simulink model "Model_MapPID_VDBTire"  (R2023a)
settings: Solver=VariableStepAuto  StartTime=0.0  StopTime=10  MaxStep=0.002  RelTol=1e-6
undefined symbols (not defined in the file): act_gain_mult, c, C_alpha_f, C_col, ctrl_delay, DiscIntNeverNeededParam, e_p0, F_zf, Iz, J_col, K, l_f, l_r, m, MapPID_H_den, MapPID_H_num, MapPID_Kaw, MapPID_Kd, MapPID_Ki, MapPID_Kp, MapPID_table, MapPID_Tf, MapPID_Ts_bp, MapPID_Ts_ctrl, MapPID_v_bp, motor_wm, n_st, noise_seed_a_y, noise_seed_gamma, noise_seed_T_s, noise_seed_theta1, noise_seed_theta2_dot, noise_seed_v, noise_var_a_y, noise_var_gamma, noise_var_T_s, noise_var_theta1, noise_var_theta2_dot, noise_var_v, sens_Tupd_a_y, sens_Tupd_gamma, sens_Tupd_T_s, sens_Tupd_theta1, sens_Tupd_theta2_dot, sens_Tupd_v, sensors_on, t_0, T_f, Tamax_table, Tamax_v_bp_ms, Tdref_ay_bp_ms2, Tdref_table, Tdref_v_bp_ms, vdb_v0
libraries: vehdynlibtire x2
settings Model: Creator=Tan_Tram  LastModifiedBy=Tan_Tram
settings DataIOCC: ReturnWorkspaceOutputs=off

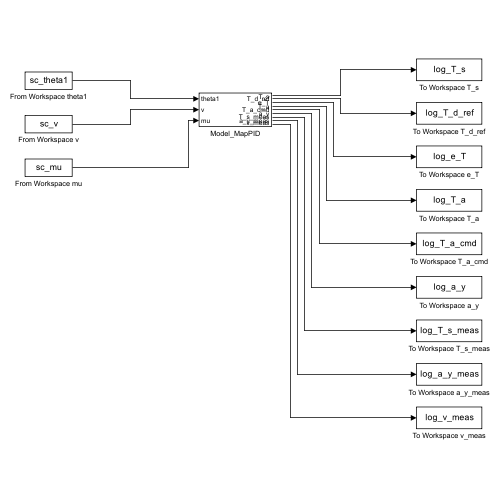
[thumbnail: Simulink's stored preview of the top-level diagram]
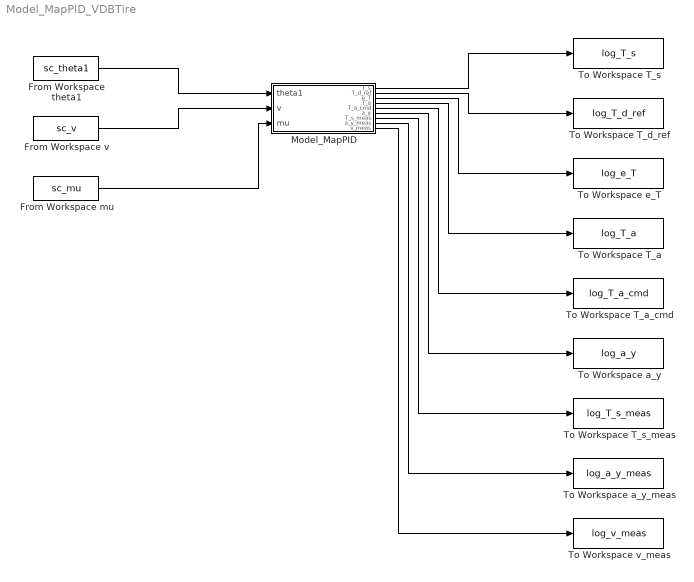
== system Model_MapPID_VDBTire ==
  From Workspace mu : FromWorkspace  VariableName=sc_mu  OutputAfterFinalValue=Holding final value
  From Workspace theta1 : FromWorkspace  VariableName=sc_theta1  OutputAfterFinalValue=Holding final value
  From Workspace v : FromWorkspace  VariableName=sc_v  OutputAfterFinalValue=Holding final value
  Model_MapPID : Subsystem
  To Workspace T_a : ToWorkspace  VariableName=log_T_a  SaveFormat=Timeseries  SampleTime=-1
  To Workspace T_a_cmd : ToWorkspace  VariableName=log_T_a_cmd  SaveFormat=Timeseries  SampleTime=-1
  To Workspace T_d_ref : ToWorkspace  VariableName=log_T_d_ref  SaveFormat=Timeseries  SampleTime=-1
  To Workspace T_s : ToWorkspace  VariableName=log_T_s  SaveFormat=Timeseries  SampleTime=-1
  To Workspace T_s_meas : ToWorkspace  VariableName=log_T_s_meas  SaveFormat=Timeseries  SampleTime=-1
  To Workspace a_y : ToWorkspace  VariableName=log_a_y  SaveFormat=Timeseries  SampleTime=-1
  To Workspace a_y_meas : ToWorkspace  VariableName=log_a_y_meas  SaveFormat=Timeseries  SampleTime=-1
  To Workspace e_T : ToWorkspace  VariableName=log_e_T  SaveFormat=Timeseries  SampleTime=-1
  To Workspace v_meas : ToWorkspace  VariableName=log_v_meas  SaveFormat=Timeseries  SampleTime=-1
  wires:
  From Workspace theta1/1 -> Model_MapPID/1(theta1)
  From Workspace v/1 -> Model_MapPID/2(v)
  From Workspace mu/1 -> Model_MapPID/3(mu)
  Model_MapPID/1(T_s) -> To Workspace T_s/1
  Model_MapPID/2(T_d_ref) -> To Workspace T_d_ref/1
  Model_MapPID/3(e_T) -> To Workspace e_T/1
  Model_MapPID/4(T_a) -> To Workspace T_a/1
  Model_MapPID/5(T_a_cmd) -> To Workspace T_a_cmd/1
  Model_MapPID/6(a_y) -> To Workspace a_y/1
  Model_MapPID/7(T_s_meas) -> To Workspace T_s_meas/1
  Model_MapPID/8(a_y_meas) -> To Workspace a_y_meas/1
  Model_MapPID/9(v_meas) -> To Workspace v_meas/1

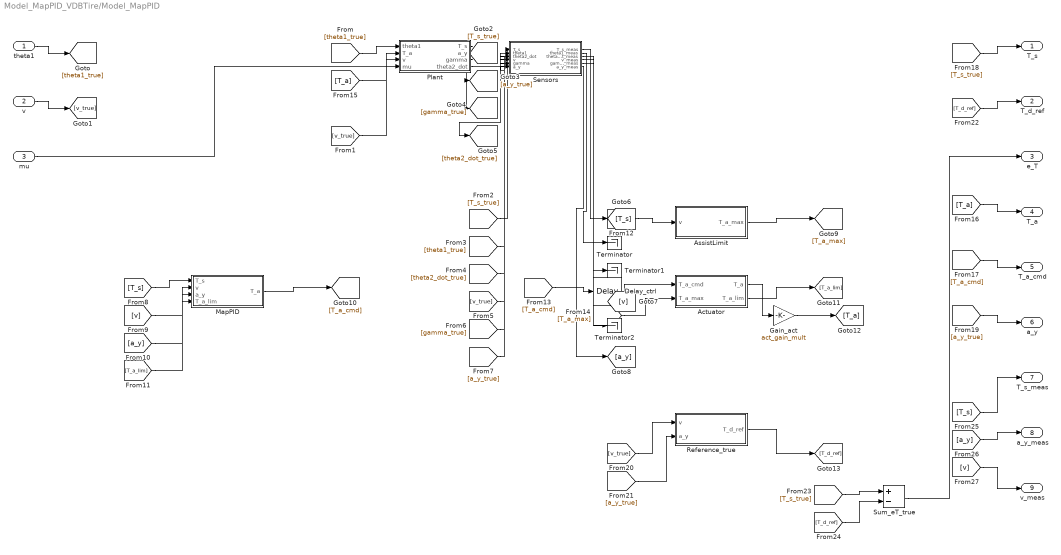
== system Model_MapPID_VDBTire/Model_MapPID ==
  theta1 : Inport
  v : Inport  Port=2
  mu : Inport  Port=3
  Actuator : Subsystem
  AssistLimit : Subsystem
  Delay_ctrl : TransportDelay  DelayTime=ctrl_delay
  Gain_act : Gain  Gain=act_gain_mult
  MapPID : Subsystem
  Plant : Subsystem
  Reference_true : Subsystem
  Sensors : Subsystem
  Sum_eT_true : Sum  Inputs=+-
  Terminator : Terminator
  Terminator1 : Terminator
  Terminator2 : Terminator
  T_s : Outport
  T_d_ref : Outport  Port=2
  e_T : Outport  Port=3
  T_a : Outport  Port=4
  T_a_cmd : Outport  Port=5
  a_y : Outport  Port=6
  T_s_meas : Outport  Port=7
  a_y_meas : Outport  Port=8
  v_meas : Outport  Port=9
  wires:
  theta1/1 -> [theta1_true]
  v/1 -> [v_true]
  mu/1 -> Plant/4(mu)
  [theta1_true] -> Plant/1(theta1)
  [v_true] -> Plant/3(v)
  Plant/1(T_s) -> [T_s_true]
  Plant/2(a_y) -> [a_y_true]
  Plant/3(gamma) -> [gamma_true]
  Plant/4(theta2_dot) -> [theta2_dot_true]
  [T_s_true] -> Sensors/1(T_s)
  [theta1_true] -> Sensors/2(theta1)
  [theta2_dot_true] -> Sensors/3(theta2_dot)
  [v_true] -> Sensors/4(v)
  [gamma_true] -> Sensors/5(gamma)
  [a_y_true] -> Sensors/6(a_y)
  Sensors/1(T_s_meas) -> [T_s]
  Sensors/2(theta1_meas) -> Terminator/1
  Sensors/3(theta2_dot_meas) -> Terminator1/1
  Sensors/4(v_meas) -> [v]
  Sensors/5(gamma_meas) -> Terminator2/1
  Sensors/6(a_y_meas) -> [a_y]
  [T_s] -> MapPID/1(T_s)
  [v] -> MapPID/2(v)
  [a_y] -> MapPID/3(a_y)
  [T_a_lim] -> MapPID/4(T_a_lim)
  [v] -> AssistLimit/1(v)
  AssistLimit/1(T_a_max) -> [T_a_max]
  MapPID/1(T_a) -> [T_a_cmd]
  [T_a_cmd] -> Delay_ctrl/1
  Delay_ctrl/1 -> Actuator/1(T_a_cmd)
  [T_a_max] -> Actuator/2(T_a_max)
  Actuator/2(T_a_lim) -> [T_a_lim]
  Actuator/1(T_a) -> Gain_act/1
  Gain_act/1 -> [T_a]
  [T_a] -> Plant/2(T_a)
  [T_a] -> T_a/1
  [T_a_cmd] -> T_a_cmd/1
  [T_s_true] -> T_s/1
  [a_y_true] -> a_y/1
  [v_true] -> Reference_true/1(v)
  [a_y_true] -> Reference_true/2(a_y)
  Reference_true/1(T_d_ref) -> [T_d_ref]
  [T_d_ref] -> T_d_ref/1
  [T_s_true] -> Sum_eT_true/1
  [T_d_ref] -> Sum_eT_true/2
  Sum_eT_true/1 -> e_T/1
  [T_s] -> T_s_meas/1
  [a_y] -> a_y_meas/1
  [v] -> v_meas/1

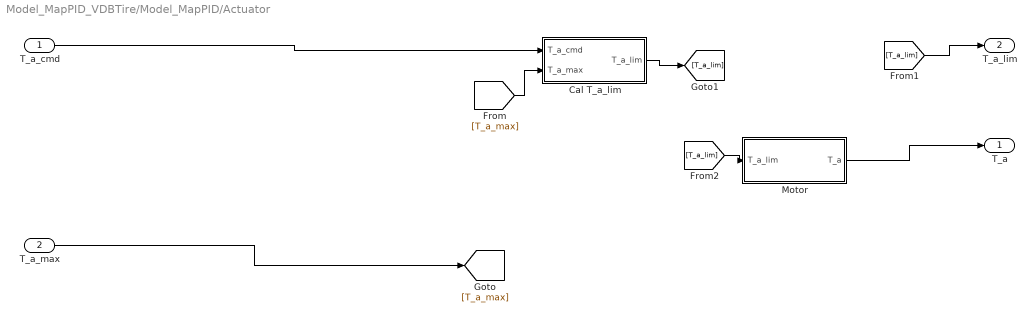
== system Model_MapPID_VDBTire/Model_MapPID/Actuator ==
  T_a_cmd : Inport
  T_a_max : Inport  Port=2
  Cal T_a_lim : Subsystem
  Motor : Subsystem
  T_a : Outport
  T_a_lim : Outport  Port=2
  wires:
  Motor/1(T_a) -> T_a/1
  [T_a_lim] -> Motor/1(T_a_lim)
  [T_a_lim] -> T_a_lim/1
  Cal T_a_lim/1(T_a_lim) -> [T_a_lim]
  [T_a_max] -> Cal T_a_lim/2(T_a_max)
  T_a_cmd/1 -> Cal T_a_lim/1(T_a_cmd)
  T_a_max/1 -> [T_a_max]

== system Model_MapPID_VDBTire/Model_MapPID/AssistLimit ==
  v : Inport
  Lookup_Tamax : Lookup_n-D  NumberOfTableDimensions=1  BreakpointsForDimension1=Tamax_v_bp_ms  Table=Tamax_table  ExtrapMethod=Clip  InternalRulePriority=Speed  RndMeth=Simplest
  T_a_max : Outport
  wires:
  Lookup_Tamax/1 -> T_a_max/1
  v/1 -> Lookup_Tamax/1

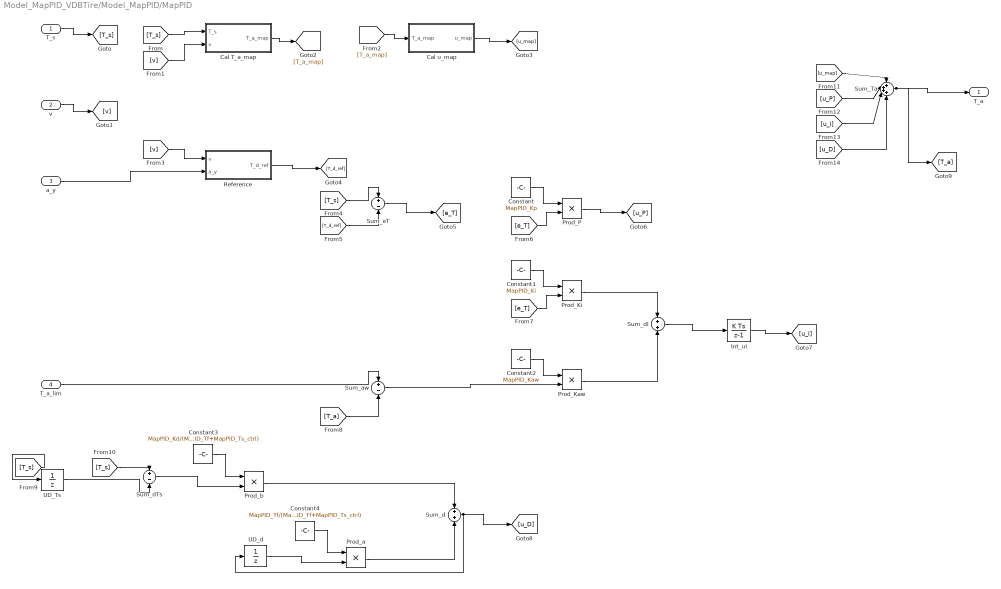
== system Model_MapPID_VDBTire/Model_MapPID/MapPID ==
  T_s : Inport
  v : Inport  Port=2
  a_y : Inport  Port=3
  T_a_lim : Inport  Port=4
  Cal T_a_map : Subsystem
  Cal u_map : Subsystem
  Constant : Constant  Value=MapPID_Kp
  Constant1 : Constant  Value=MapPID_Ki
  Constant2 : Constant  Value=MapPID_Kaw
  Constant3 : Constant  Value=MapPID_Kd/(MapPID_Tf+MapPID_Ts_ctrl)
  Constant4 : Constant  Value=MapPID_Tf/(MapPID_Tf+MapPID_Ts_ctrl)
  Int_uI : DiscreteIntegrator  gainval=1  SampleTime=MapPID_Ts_ctrl  ICPrevOutput=DiscIntNeverNeededParam  ICPrevScaledInput=DiscIntNeverNeededParam
  Prod_Kaw : Product  Inputs=**
  Prod_Ki : Product  Inputs=**
  Prod_P : Product  Inputs=**
  Prod_a : Product  Inputs=**
  Prod_b : Product  Inputs=**
  Reference : Subsystem
  Sum_Ta : Sum  Inputs=++++
  Sum_aw : Sum  Inputs=+-
  Sum_d : Sum
  Sum_dI : Sum
  Sum_dTs : Sum  Inputs=+-
  Sum_eT : Sum  Inputs=+-
  UD_Ts : UnitDelay  SampleTime=MapPID_Ts_ctrl  HasFrameUpgradeWarning=on
  UD_d : UnitDelay  SampleTime=MapPID_Ts_ctrl  HasFrameUpgradeWarning=on
  T_a : Outport
  wires:
  Sum_Ta/1 -> [T_a], T_a/1
  [u_D] -> Sum_Ta/4
  [u_I] -> Sum_Ta/3
  [u_P] -> Sum_Ta/2
  [u_map] -> Sum_Ta/1
  Sum_d/1 -> [u_D], UD_d/1
  Prod_a/1 -> Sum_d/2
  Prod_b/1 -> Sum_d/1
  UD_d/1 -> Prod_a/2
  Constant4/1 -> Prod_a/1
  Sum_dTs/1 -> Prod_b/2
  Constant3/1 -> Prod_b/1
  UD_Ts/1 -> Sum_dTs/2
  [T_s] -> Sum_dTs/1
  [T_s] -> UD_Ts/1
  Int_uI/1 -> [u_I]
  Sum_dI/1 -> Int_uI/1
  Prod_Kaw/1 -> Sum_dI/2
  Prod_Ki/1 -> Sum_dI/1
  Sum_aw/1 -> Prod_Kaw/2
  Constant2/1 -> Prod_Kaw/1
  [T_a] -> Sum_aw/2
  T_a_lim/1 -> Sum_aw/1
  [e_T] -> Prod_Ki/2
  Constant1/1 -> Prod_Ki/1
  Prod_P/1 -> [u_P]
  [e_T] -> Prod_P/2
  Constant/1 -> Prod_P/1
  Sum_eT/1 -> [e_T]
  [T_d_ref] -> Sum_eT/2
  [T_s] -> Sum_eT/1
  Reference/1(T_d_ref) -> [T_d_ref]
  a_y/1 -> Reference/2(a_y)
  [v] -> Reference/1(v)
  Cal u_map/1(u_map) -> [u_map]
  [T_a_map] -> Cal u_map/1(T_a_map)
  Cal T_a_map/1(T_a_map) -> [T_a_map]
  [v] -> Cal T_a_map/2(v)
  [T_s] -> Cal T_a_map/1(T_s)
  v/1 -> [v]
  T_s/1 -> [T_s]

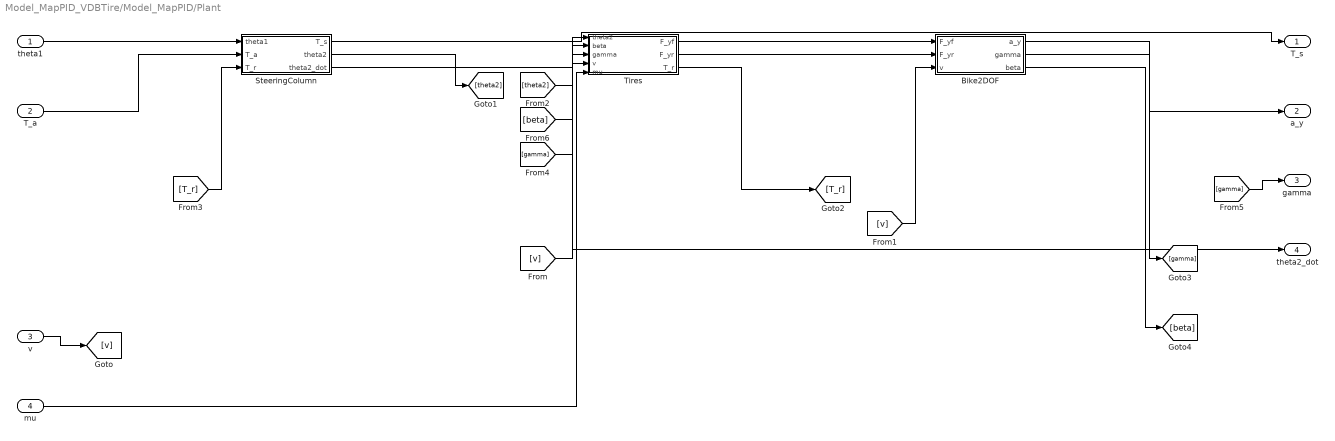
== system Model_MapPID_VDBTire/Model_MapPID/Plant ==
  theta1 : Inport
  T_a : Inport  Port=2
  v : Inport  Port=3
  mu : Inport  Port=4
  Bike2DOF : Subsystem
  SteeringColumn : Subsystem
  Tires : Subsystem
  T_s : Outport
  a_y : Outport  Port=2
  gamma : Outport  Port=3
  theta2_dot : Outport  Port=4
  wires:
  theta1/1 -> SteeringColumn/1(theta1)
  T_a/1 -> SteeringColumn/2(T_a)
  mu/1 -> Tires/5(mu)
  Tires/1(F_yf) -> Bike2DOF/1(F_yf)
  Tires/2(F_yr) -> Bike2DOF/2(F_yr)
  SteeringColumn/1(T_s) -> T_s/1
  Bike2DOF/1(a_y) -> a_y/1
  SteeringColumn/3(theta2_dot) -> theta2_dot/1
  v/1 -> [v]
  [v] -> Tires/4(v)
  [v] -> Bike2DOF/3(v)
  SteeringColumn/2(theta2) -> [theta2]
  [theta2] -> Tires/1(theta2)
  Tires/3(T_r) -> [T_r]
  [T_r] -> SteeringColumn/3(T_r)
  Bike2DOF/2(gamma) -> [gamma]
  [gamma] -> Tires/3(gamma)
  [gamma] -> gamma/1
  Bike2DOF/3(beta) -> [beta]
  [beta] -> Tires/2(beta)

== system Model_MapPID_VDBTire/Model_MapPID/Reference_true ==
  v : Inport
  a_y : Inport  Port=2
  Cal T_d_ref : Subsystem
  T_d_ref : Outport
  wires:
  Cal T_d_ref/1(T_d_ref) -> T_d_ref/1
  a_y/1 -> Cal T_d_ref/2(a_y)
  v/1 -> Cal T_d_ref/1(v)

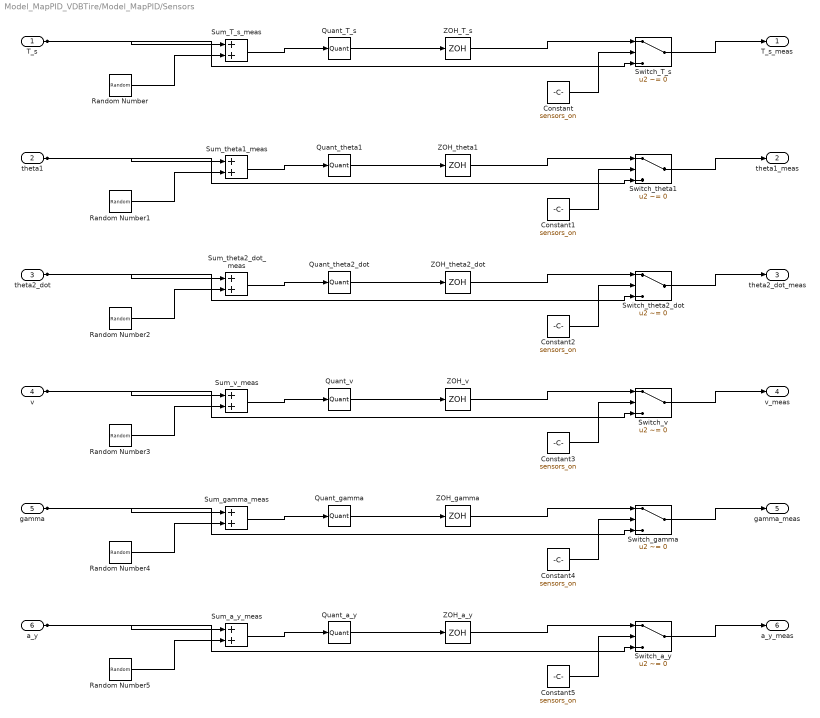
== system Model_MapPID_VDBTire/Model_MapPID/Sensors ==
  T_s : Inport
  theta1 : Inport  Port=2
  theta2_dot : Inport  Port=3
  v : Inport  Port=4
  gamma : Inport  Port=5
  a_y : Inport  Port=6
  Constant{,1..5} (6 alike) : Constant  Value=sensors_on
  Quant_T_s : Quantizer  QuantizationInterval=sens_delta_T_s
  Quant_a_y : Quantizer  QuantizationInterval=sens_delta_a_y
  Quant_gamma : Quantizer  QuantizationInterval=sens_delta_gamma
  Quant_theta1 : Quantizer  QuantizationInterval=sens_delta_theta1
  Quant_theta2_dot : Quantizer  QuantizationInterval=sens_delta_theta2_dot
  Quant_v : Quantizer  QuantizationInterval=sens_delta_v
  Random Number : RandomNumber  Variance=noise_var_T_s  Seed=noise_seed_T_s  SampleTime=sens_Tupd_T_s
  Random Number1 : RandomNumber  Variance=noise_var_theta1  Seed=noise_seed_theta1  SampleTime=sens_Tupd_theta1
  Random Number2 : RandomNumber  Variance=noise_var_theta2_dot  Seed=noise_seed_theta2_dot  SampleTime=sens_Tupd_theta2_dot
  Random Number3 : RandomNumber  Variance=noise_var_v  Seed=noise_seed_v  SampleTime=sens_Tupd_v
  Random Number4 : RandomNumber  Variance=noise_var_gamma  Seed=noise_seed_gamma  SampleTime=sens_Tupd_gamma
  Random Number5 : RandomNumber  Variance=noise_var_a_y  Seed=noise_seed_a_y  SampleTime=sens_Tupd_a_y
  Sum_T_s_meas : Sum
  Sum_a_y_meas : Sum
  Sum_gamma_meas : Sum
  Sum_theta1_meas : Sum
  Sum_theta2_dot_meas : Sum
  Sum_v_meas : Sum
  Switch_T_s : Switch  Criteria=u2 ~= 0  SaturateOnIntegerOverflow=off  InputSameDT=off
  Switch_a_y : Switch  Criteria=u2 ~= 0  SaturateOnIntegerOverflow=off  InputSameDT=off
  Switch_gamma : Switch  Criteria=u2 ~= 0  SaturateOnIntegerOverflow=off  InputSameDT=off
  Switch_theta1 : Switch  Criteria=u2 ~= 0  SaturateOnIntegerOverflow=off  InputSameDT=off
  Switch_theta2_dot : Switch  Criteria=u2 ~= 0  SaturateOnIntegerOverflow=off  InputSameDT=off
  Switch_v : Switch  Criteria=u2 ~= 0  SaturateOnIntegerOverflow=off  InputSameDT=off
  ZOH_T_s : ZeroOrderHold  SampleTime=sens_Tupd_T_s
  ZOH_a_y : ZeroOrderHold  SampleTime=sens_Tupd_a_y
  ZOH_gamma : ZeroOrderHold  SampleTime=sens_Tupd_gamma
  ZOH_theta1 : ZeroOrderHold  SampleTime=sens_Tupd_theta1
  ZOH_theta2_dot : ZeroOrderHold  SampleTime=sens_Tupd_theta2_dot
  ZOH_v : ZeroOrderHold  SampleTime=sens_Tupd_v
  T_s_meas : Outport
  theta1_meas : Outport  Port=2
  theta2_dot_meas : Outport  Port=3
  v_meas : Outport  Port=4
  gamma_meas : Outport  Port=5
  a_y_meas : Outport  Port=6
  wires:
  Switch_a_y/1 -> a_y_meas/1
  Constant5/1 -> Switch_a_y/2
  ZOH_a_y/1 -> Switch_a_y/1
  Quant_a_y/1 -> ZOH_a_y/1
  Sum_a_y_meas/1 -> Quant_a_y/1
  Random Number5/1 -> Sum_a_y_meas/2
  a_y/1 -> Switch_a_y/3, Sum_a_y_meas/1
  Switch_gamma/1 -> gamma_meas/1
  Constant4/1 -> Switch_gamma/2
  ZOH_gamma/1 -> Switch_gamma/1
  Quant_gamma/1 -> ZOH_gamma/1
  Sum_gamma_meas/1 -> Quant_gamma/1
  Random Number4/1 -> Sum_gamma_meas/2
  gamma/1 -> Switch_gamma/3, Sum_gamma_meas/1
  Switch_v/1 -> v_meas/1
  Constant3/1 -> Switch_v/2
  ZOH_v/1 -> Switch_v/1
  Quant_v/1 -> ZOH_v/1
  Sum_v_meas/1 -> Quant_v/1
  Random Number3/1 -> Sum_v_meas/2
  v/1 -> Switch_v/3, Sum_v_meas/1
  Switch_theta2_dot/1 -> theta2_dot_meas/1
  Constant2/1 -> Switch_theta2_dot/2
  ZOH_theta2_dot/1 -> Switch_theta2_dot/1
  Quant_theta2_dot/1 -> ZOH_theta2_dot/1
  Sum_theta2_dot_meas/1 -> Quant_theta2_dot/1
  Random Number2/1 -> Sum_theta2_dot_meas/2
  theta2_dot/1 -> Switch_theta2_dot/3, Sum_theta2_dot_meas/1
  Switch_theta1/1 -> theta1_meas/1
  Constant1/1 -> Switch_theta1/2
  ZOH_theta1/1 -> Switch_theta1/1
  Quant_theta1/1 -> ZOH_theta1/1
  Sum_theta1_meas/1 -> Quant_theta1/1
  Random Number1/1 -> Sum_theta1_meas/2
  theta1/1 -> Switch_theta1/3, Sum_theta1_meas/1
  Switch_T_s/1 -> T_s_meas/1
  Constant/1 -> Switch_T_s/2
  ZOH_T_s/1 -> Switch_T_s/1
  Quant_T_s/1 -> ZOH_T_s/1
  Sum_T_s_meas/1 -> Quant_T_s/1
  Random Number/1 -> Sum_T_s_meas/2
  T_s/1 -> Switch_T_s/3, Sum_T_s_meas/1

== system Model_MapPID_VDBTire/Model_MapPID/Actuator/Cal T_a_lim ==
  T_a_cmd : Inport
  T_a_max : Inport  Port=2
  Max_Ta : MinMax  Function=max  Inputs=2
  Min_Ta : MinMax  Inputs=2
  Neg_Tamax : UnaryMinus
  T_a_lim : Outport
  wires:
  Max_Ta/1 -> T_a_lim/1
  Neg_Tamax/1 -> Max_Ta/2
  Min_Ta/1 -> Max_Ta/1
  [T_a_max] -> Neg_Tamax/1
  [T_a_max] -> Min_Ta/2
  T_a_cmd/1 -> Min_Ta/1
  T_a_max/1 -> [T_a_max]

== system Model_MapPID_VDBTire/Model_MapPID/Actuator/Motor ==
  T_a_lim : Inport
  Motor_lag : TransferFcn  Numerator=[motor_wm]  Denominator=[1 motor_wm]
  T_a : Outport
  wires:
  Motor_lag/1 -> T_a/1
  T_a_lim/1 -> Motor_lag/1

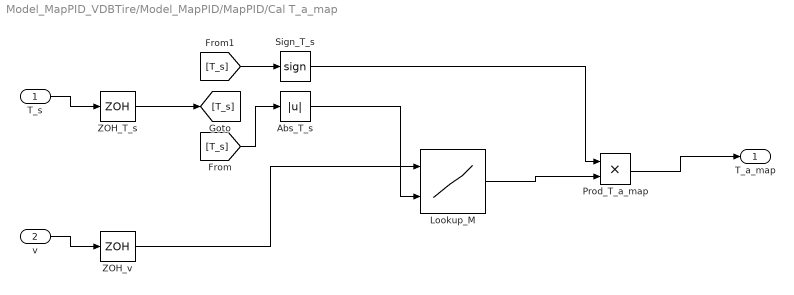
== system Model_MapPID_VDBTire/Model_MapPID/MapPID/Cal T_a_map ==
  T_s : Inport
  v : Inport  Port=2
  Abs_T_s : Abs  SaturateOnIntegerOverflow=off
  Lookup_M : Lookup_n-D  BreakpointsForDimension1=MapPID_v_bp  BreakpointsForDimension2=MapPID_Ts_bp  BreakpointsForDimension3=[5, 7]  Table=MapPID_table  ExtrapMethod=Clip  InternalRulePriority=Speed  RndMeth=Simplest
      settings: InputPortMap=u0,u1
  Prod_T_a_map : Product  Inputs=**
  Sign_T_s : Signum
  ZOH_T_s : ZeroOrderHold  SampleTime=MapPID_Ts_ctrl
  ZOH_v : ZeroOrderHold  SampleTime=MapPID_Ts_ctrl
  T_a_map : Outport
  wires:
  Prod_T_a_map/1 -> T_a_map/1
  Lookup_M/1 -> Prod_T_a_map/2
  Sign_T_s/1 -> Prod_T_a_map/1
  Abs_T_s/1 -> Lookup_M/2
  ZOH_v/1 -> Lookup_M/1
  [T_s] -> Sign_T_s/1
  [T_s] -> Abs_T_s/1
  ZOH_T_s/1 -> [T_s]
  v/1 -> ZOH_v/1
  T_s/1 -> ZOH_T_s/1

== system Model_MapPID_VDBTire/Model_MapPID/MapPID/Cal u_map ==
  T_a_map : Inport
  Disc_H : DiscreteTransferFcn  Numerator=MapPID_H_num  Denominator=MapPID_H_den  SampleTime=MapPID_Ts_ctrl
  u_map : Outport
  wires:
  Disc_H/1 -> u_map/1
  [T_a_map] -> Disc_H/1
  T_a_map/1 -> [T_a_map]

== system Model_MapPID_VDBTire/Model_MapPID/MapPID/Reference ==
  v : Inport
  a_y : Inport  Port=2
  Cal T_d_ref : Subsystem
  T_d_ref : Outport
  wires:
  v/1 -> Cal T_d_ref/1(v)
  a_y/1 -> Cal T_d_ref/2(a_y)
  Cal T_d_ref/1(T_d_ref) -> T_d_ref/1

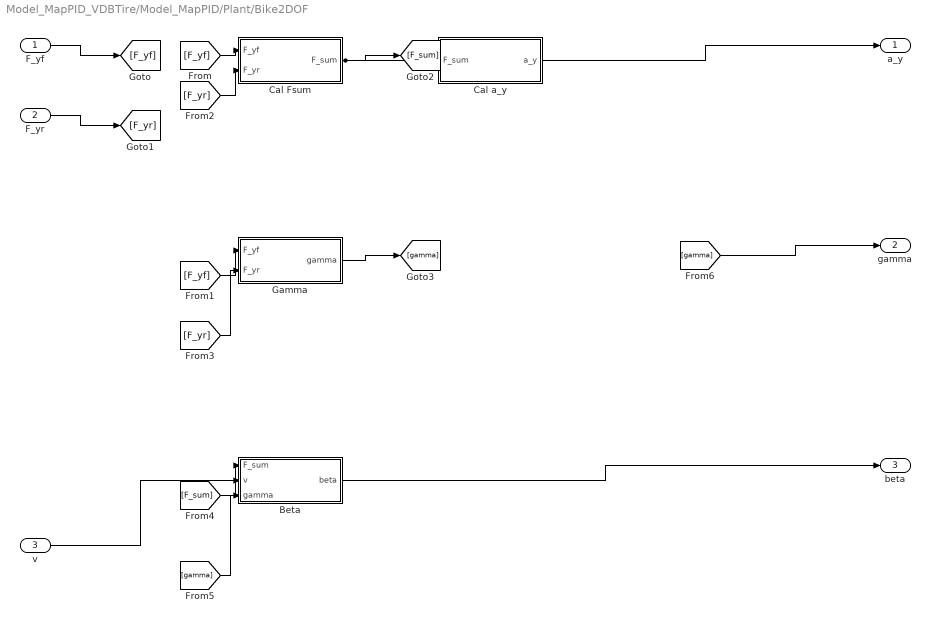
== system Model_MapPID_VDBTire/Model_MapPID/Plant/Bike2DOF ==
  F_yf : Inport
  F_yr : Inport  Port=2
  v : Inport  Port=3
  Beta : Subsystem
  Cal Fsum : Subsystem
  Cal a_y : Subsystem
  Gamma : Subsystem
  a_y : Outport
  gamma : Outport  Port=2
  beta : Outport  Port=3
  wires:
  Beta/1(beta) -> beta/1
  v/1 -> Beta/2(v)
  [gamma] -> gamma/1
  [gamma] -> Beta/3(gamma)
  Gamma/1(gamma) -> [gamma]
  Cal a_y/1(a_y) -> a_y/1
  [F_sum] -> Beta/1(F_sum)
  Cal Fsum/1(F_sum) -> [F_sum], Cal a_y/1(F_sum)
  [F_yr] -> Gamma/2(F_yr)
  [F_yr] -> Cal Fsum/2(F_yr)
  F_yr/1 -> [F_yr]
  [F_yf] -> Gamma/1(F_yf)
  [F_yf] -> Cal Fsum/1(F_yf)
  F_yf/1 -> [F_yf]

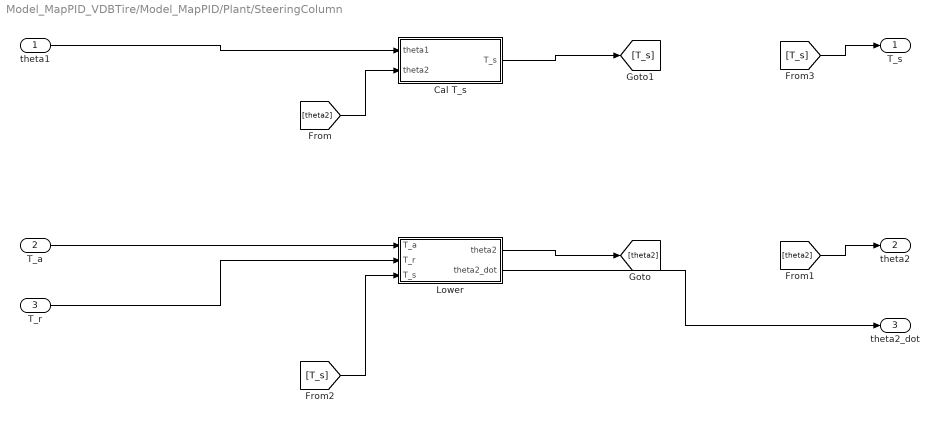
== system Model_MapPID_VDBTire/Model_MapPID/Plant/SteeringColumn ==
  theta1 : Inport
  T_a : Inport  Port=2
  T_r : Inport  Port=3
  Cal T_s : Subsystem
  Lower : Subsystem
  T_s : Outport
  theta2 : Outport  Port=2
  theta2_dot : Outport  Port=3
  wires:
  [T_s] -> T_s/1
  [T_s] -> Lower/3(T_s)
  Cal T_s/1(T_s) -> [T_s]
  [theta2] -> theta2/1
  [theta2] -> Cal T_s/2(theta2)
  Lower/1(theta2) -> [theta2]
  Lower/2(theta2_dot) -> theta2_dot/1
  T_r/1 -> Lower/2(T_r)
  T_a/1 -> Lower/1(T_a)
  theta1/1 -> Cal T_s/1(theta1)

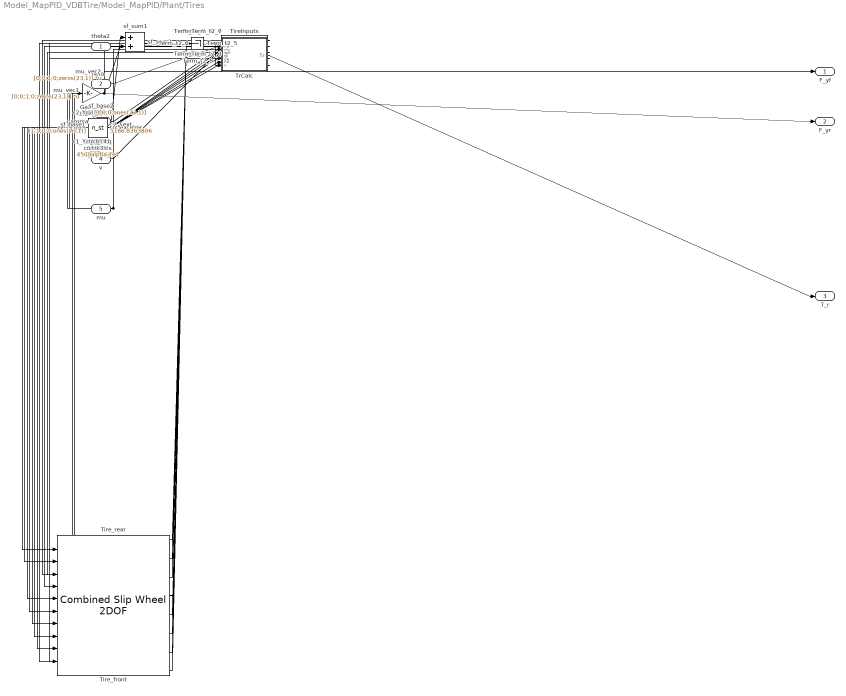
== system Model_MapPID_VDBTire/Model_MapPID/Plant/Tires ==
  theta2 : Inport
  beta : Inport  Port=2
  gamma : Inport  Port=3
  v : Inport  Port=4
  mu : Inport  Port=5
  Gain_F1 : Gain  Gain=2
  Gain_F2 : Gain  Gain=2
  Term_t1_{1..3,5..8} (7 alike) : Terminator
  Term_t2_{1..3,5..8} (7 alike) : Terminator
  TireInputs : MATLAB Function  TreatAsAtomicUnit=on
  Tire_front : vehdynlibtire/Combined Slip Wheel 2DOF  tireType=External file  BrakeType=Disc  vertType=None  plySteer=off  turnslip=off  mu_static=.3  mu_kinetic=.2  disk_abore=.05  Rm=.177  num_pads=2  drum_abore=0.0508  drum_a=0.123  drum_c=0.212  drum_r=0.15  drum_theta1=0  drum_theta2=126  brake_p_bpt=[1 11.4736842105263 21.9473684210526 32.4210526315789 42.8947368421053 53.3684210526316 63.8421052631579 74.3157894736842 84.7894736842105 95.2631578947368 105.736842105263 116.210526315789 126.684210526316 137.157894736842 147.631578947368 158.105263157895 168.578947368421 179.052631578947 189.526315789474 200]  brake_n_bpt=[0 52.6315789473684 105.263157894737 157.894736842105 210.526315789474 263.157894736842 315.789473684211 368.421052631579 421.052631578947 473.684210526316 526.315789473684 578.947368421053 631.578947368421 684.210526315789 736.842105263158 789.473684210526 842.105263157895 894.736842105263 947.368421052632 1000]  f_brake_t=[43.4900602404453 42.5056030554862 41.5350898940194 40.5780454442085 39.6340111501808 38.7025443887544 37.7832176914519 36.8756180088306 35.9793460143796 35.0940154454303 34.2192524787115 33.3546951383474 32.4999927342521 31.6548053290159 30.8188032315107 29.991666515561 29.1730845621415 28.362755623661 27.5603864089927 26.765691687993;498.991217495636 487.695866636631 476.560505099801 465.579679307235 454.748127933653 444.060772460445 433.51270824929 423.099196101319 412.81565427025 402.657650900201 392.620896861006 382.701238955775 372.894653477208 363.197240090814 353.605216024701 344.114910546964 334.722759712992 325.425301366216 316.219170376863 307.10109410434;954.492374750826 932.886130217776 911.585920305583 890.581313170261 869.862244717126 849.419000532136 829.242198807128 809.322774193808 789.651962526121 770.221286354971 751.0225412433 732.047782773203 713.289314220164 694.739674852612 676.391628817892 658.238154578366 640.272434863842 622.48784710877 604.877954344734 587.436496520688;1409.99353200602 1378.07639379892 1346.61133551136 1315.58294703329 1284.9763615006 1254.77722860383 1224.97168936497 1195.5463522863 1166.48827078199 1137.78492180974 1109.42418562559 1081.39432659063 1053.68397496312 1026.28210961441 999.178041611083 972.361398609768 945.822110014692 919.550392851325 893.536738312604 867.771898937035;1865.49468926121 1823.26665738007 1781.63675071715 1740.58458089631 1700.09047828407 1660.13545667552 1620.7011799228 1581.76993037878 1543.32457903786 1505.34855726451 1467.82583000789 1430.74087040806 1394.07863570608 1357.82454437621 1321.96445440427 1286.48464264117 1251.37178516554 1216.61293859388 1182.19552228048 1148.10730135338;2320.9958465164 2268.45692096121 2216.66216592293 2165.58621475934 2115.20459506754 2065.49368474721 2016.43067048064 1967.99350847127 1920.16088729373 1872.91219271928 1826.22747439018 1780.08741422549 1734.47329644903 1689.36697913801 1644.75086719747 1600.60788667257 1556.92146031639 1513.67548433643 1470.85430624835 1428.44270376973;2776.49700377159 2713.64718454235 2651.68758112871 2590.58784862237 2530.31871185102 2470.8519128189 2412.16016103848 2354.21708656376 2296.9971955496 2240.47582817405 2184.62911877248 2129.43395804292 2074.86795719199 2020.9094138998 1967.53727999066 1914.73113070398 1862.47113546724 1810.73803007899 1759.51309021622 1708.77810618608;3231.99816102678 3158.8374481235 3086.71299633449 3015.58948248539 2945.43282863449 2876.21014089059 2807.88965159632 2740.44066465625 2673.83350380547 2608.03946362882 2543.03076315477 2478.78050186034 2415.26261793494 2352.4518486616 2290.32369278385 2228.85437473538 2168.02081061809 2107.80057582154 2048.17187418409 1989.11350860242;3687.49931828197 3604.02771170464 3521.73841154027 3440.59111634842 3360.54694541796 3281.56836896228 3203.61914215416 3126.66424274874 3050.66981206134 2975.60309908359 2901.43240753707 2828.12704567777 2755.6572786779 2683.9942834234 2613.11010557704 2542.97761876678 2473.57048576894 2404.8631215641 2336.83065815196 2269.44891101877;4143.00047553716 4049.21797528579 3956.76382674606 3865.59275021144 3775.66106220143 3686.92659703397 3599.34863271199 3512.88782084123 3427.50612031721 3343.16673453836 3259.83405191936 3177.4735894952 3096.05193942085 3015.5367181852 2935.89651837023 2857.10086279818 2779.12016091979 2701.92566730665 2625.48944211983 2549.78431343512;4598.50163279235 4494.40823886693 4391.78924195184 4290.59438407447 4190.77517898491 4092.28482510566 3995.07812326983 3899.11139893372 3804.34242857308 3710.73036999313 3618.23569630166 3526.82013331263 3436.44660016381 3347.079152947 3258.68293116342 3171.22410682959 3084.66983607064 2998.98821304921 2914.1482260877 2830.11971585147;5054.00279004754 4939.59850244808 4826.81465715762 4715.59601793749 4605.88929576838 4497.64305317735 4390.80761382767 4285.3349770262 4181.17873682896 4078.2940054479 3976.63734068395 3876.16667713006 3776.84126090677 3678.62158770879 3581.46934395661 3485.34735086099 ...(+2764 chars)]  tireParamSet=vdynPassCar.mat  PRESMAX=1000000  PRESMIN=10000  FZMAX=28000  FZMIN=100  VXLOW=1  KPUMAX=1.5  KPUMIN=-1.5  ALPMAX=1.5  ALPMIN=-1.5  CAMMAX=0.17453  CAMMIN=-0.17453  LONGVL=16.7  FxRelFreqLwrLim=200*pi  FyRelFreqLwrLim=200*pi  MyRelFreqLwrLim=100*pi  omegao=vdb_v0/(0.97*0.5132)  br=1e-3  UNLOADED_RADIUS=0.5132  NOMPRES=793000  FNOMIN=4548.7286194  WIDTH=0.295  RIM_RADIUS=0.28575  MASS=54.96  IYY=10.664  GRAVITY=-9.81  zo=0  zdoto=0  BREFF=8.25094594147963  DREFF=0.260468730454265  FREFF=0.0735298544471851  Q_RE0=1.00866439868088  Q_V1=0.000760413786224011  Q_V2=0.0463384792019201  Q_FZ1=0  Q_FZ2=15.6870832810226  Q_FZ3=0  Q_FCX=0.138643970247602  Q_FCY=0.10843499565426  Q_FCY2=-0.465763352339538  PFZ1=0.69958166705601  VERTICAL_STIFFNESS=207885.061134007  VERTICAL_DAMPING=500  BOTTOM_OFFST=.01  BOTTOM_STIFF=2e6  LONGITUDINAL_STIFFNESS=388714.175879854  LATERAL_STIFFNESS=157087.404633332  PCFX1=0.18539229191199  PCFX2=0  PCFX3=0  PCFY1=0.163183345037677  PCFY2=0  PCFY3=0.249094918231954  Q_RA1=0.675942571700787  Q_RA2=0.73800463546164  Q_RB1=1.04487486456705  Q_RB2=-1.191763806629  PCX1=1.58523057950359  PDX1=1.0239116238178  PDX2=-0.0842405110022724  PDX3=0  PEX1=0.110312777158455  PEX2=0.313468516038146  PEX3=0  PEX4=0.0016060905760045  PKX1=21.3872544684023  PKX2=14.0006541873175  PKX3=-0.405326109653452  PHX1=0.000212599305364818  PHX2=0.00115950515263055  PVX1=1.59236164471432e-05  PVX2=0.000104321112127671  PPX1=-0.349461321276586  PPX2=0.387840040616429  PPX3=-0.0969947336569324  PPX4=0.0632271859795801  RBX1=12.7633329850276  RBX2=9.5787123658471  RBX3=0  RCX1=1.02796280922059  REX1=-0.45202516851367  REX2=-0.47304886171176  RHX1=0.000233272373115809  QSX1=-0.00788307788961443  QSX2=0.954629515459396  QSX3=0.0155855777667025  QSX4=0.125904607142414  QSX5=1.01110069703963  QSX6=20.1938577118433  QSX7=0.310818120717083  QSX8=-0.0430823751139655  QSX9=0.636494404888216  QSX10=0.142438060591663  QSX11=0.346766530036373  QSX12=0  QSX13=0  QSX14=0  PPMX1=0  PCY1=1.3  PDY1=1  PDY2=0  PDY3=0  PEY1=-1  PEY2=0  PEY3=0  PEY4=0  PEY5=0  PKY1=-17.5873319104  PKY2=1  PKY3=0  PKY4=2  PKY5=0  PKY6=0  PKY7=0  PHY1=0  PHY2=0  PVY1=0  PVY2=0  PVY3=0  PVY4=0  PPY1=0  PPY2=0  PPY3=0  PPY4=0  PPY5=0  RBY1=0  RBY2=0  RBY3=0  RBY4=0  RCY1=1  REY1=0  REY2=0  RHY1=0  RHY2=0  RVY1=0  RVY2=0  RVY3=0  RVY4=0  RVY5=0  RVY6=0  QSY1=0  QSY2=0  QSY3=0  QSY4=0  QSY5=0  QSY6=0  QSY7=0  QSY8=0  QBZ1=11.666656027484  QBZ2=-1.30355438574485  QBZ3=0  QBZ4=0.177918305399071  QBZ5=-0.162481135068033  QBZ6=0  QBZ9=30.1445534682089  QBZ10=0  QCZ1=1.29026978207574  QDZ1=0.0886972644991399  QDZ2=-0.0058634820161856  QDZ3=0.3805597481383  QDZ4=0  QDZ6=0.00160914918118959  QDZ7=-0.00211036330862154  QDZ8=-0.13921904912557  QDZ9=0.00816585550028243  QDZ10=0  QDZ11=0  QEZ1=-2.19802254534746  QEZ2=1.01850535789165  QEZ3=0  QEZ4=0.278379679112054  QEZ5=-0.548414722765386  QHZ1=0.00148361198869669  QHZ2=0.00202017567585904  QHZ3=0.240316641332066  QHZ4=-0.210114035738085  PPZ1=-0.443927982388615  PPZ2=0  SSZ1=0.00914999585397887  SSZ2=0.0389830656052735  SSZ3=0  SSZ4=0  PDXP1=0.396718274678791  PDXP2=0  PDXP3=0  PKYP1=1.00587060633573  PDYP1=0.40483048923438  PDYP2=0  PDYP3=0  PDYP4=0  PHYP1=0.992731942067188  PHYP2=0.150352945499914  PHYP3=0  PHYP4=-3.98988682633674  PECP1=0.502379254513503  PECP2=0  QDTP1=10.0178654287947  QCRP1=0.200627747200702  QCRP2=0.0995735881599772  QBRP1=0.0997107127960717  QDRP1=1.01432910167423  QDRP2=0  aMode=2
  Tire_rear : vehdynlibtire/Combined Slip Wheel 2DOF  tireType=External file  BrakeType=Disc  vertType=None  plySteer=off  turnslip=off  mu_static=.3  mu_kinetic=.2  disk_abore=.05  Rm=.177  num_pads=2  drum_abore=0.0508  drum_a=0.123  drum_c=0.212  drum_r=0.15  drum_theta1=0  drum_theta2=126  brake_p_bpt=[1 11.4736842105263 21.9473684210526 32.4210526315789 42.8947368421053 53.3684210526316 63.8421052631579 74.3157894736842 84.7894736842105 95.2631578947368 105.736842105263 116.210526315789 126.684210526316 137.157894736842 147.631578947368 158.105263157895 168.578947368421 179.052631578947 189.526315789474 200]  brake_n_bpt=[0 52.6315789473684 105.263157894737 157.894736842105 210.526315789474 263.157894736842 315.789473684211 368.421052631579 421.052631578947 473.684210526316 526.315789473684 578.947368421053 631.578947368421 684.210526315789 736.842105263158 789.473684210526 842.105263157895 894.736842105263 947.368421052632 1000]  f_brake_t=[43.4900602404453 42.5056030554862 41.5350898940194 40.5780454442085 39.6340111501808 38.7025443887544 37.7832176914519 36.8756180088306 35.9793460143796 35.0940154454303 34.2192524787115 33.3546951383474 32.4999927342521 31.6548053290159 30.8188032315107 29.991666515561 29.1730845621415 28.362755623661 27.5603864089927 26.765691687993;498.991217495636 487.695866636631 476.560505099801 465.579679307235 454.748127933653 444.060772460445 433.51270824929 423.099196101319 412.81565427025 402.657650900201 392.620896861006 382.701238955775 372.894653477208 363.197240090814 353.605216024701 344.114910546964 334.722759712992 325.425301366216 316.219170376863 307.10109410434;954.492374750826 932.886130217776 911.585920305583 890.581313170261 869.862244717126 849.419000532136 829.242198807128 809.322774193808 789.651962526121 770.221286354971 751.0225412433 732.047782773203 713.289314220164 694.739674852612 676.391628817892 658.238154578366 640.272434863842 622.48784710877 604.877954344734 587.436496520688;1409.99353200602 1378.07639379892 1346.61133551136 1315.58294703329 1284.9763615006 1254.77722860383 1224.97168936497 1195.5463522863 1166.48827078199 1137.78492180974 1109.42418562559 1081.39432659063 1053.68397496312 1026.28210961441 999.178041611083 972.361398609768 945.822110014692 919.550392851325 893.536738312604 867.771898937035;1865.49468926121 1823.26665738007 1781.63675071715 1740.58458089631 1700.09047828407 1660.13545667552 1620.7011799228 1581.76993037878 1543.32457903786 1505.34855726451 1467.82583000789 1430.74087040806 1394.07863570608 1357.82454437621 1321.96445440427 1286.48464264117 1251.37178516554 1216.61293859388 1182.19552228048 1148.10730135338;2320.9958465164 2268.45692096121 2216.66216592293 2165.58621475934 2115.20459506754 2065.49368474721 2016.43067048064 1967.99350847127 1920.16088729373 1872.91219271928 1826.22747439018 1780.08741422549 1734.47329644903 1689.36697913801 1644.75086719747 1600.60788667257 1556.92146031639 1513.67548433643 1470.85430624835 1428.44270376973;2776.49700377159 2713.64718454235 2651.68758112871 2590.58784862237 2530.31871185102 2470.8519128189 2412.16016103848 2354.21708656376 2296.9971955496 2240.47582817405 2184.62911877248 2129.43395804292 2074.86795719199 2020.9094138998 1967.53727999066 1914.73113070398 1862.47113546724 1810.73803007899 1759.51309021622 1708.77810618608;3231.99816102678 3158.8374481235 3086.71299633449 3015.58948248539 2945.43282863449 2876.21014089059 2807.88965159632 2740.44066465625 2673.83350380547 2608.03946362882 2543.03076315477 2478.78050186034 2415.26261793494 2352.4518486616 2290.32369278385 2228.85437473538 2168.02081061809 2107.80057582154 2048.17187418409 1989.11350860242;3687.49931828197 3604.02771170464 3521.73841154027 3440.59111634842 3360.54694541796 3281.56836896228 3203.61914215416 3126.66424274874 3050.66981206134 2975.60309908359 2901.43240753707 2828.12704567777 2755.6572786779 2683.9942834234 2613.11010557704 2542.97761876678 2473.57048576894 2404.8631215641 2336.83065815196 2269.44891101877;4143.00047553716 4049.21797528579 3956.76382674606 3865.59275021144 3775.66106220143 3686.92659703397 3599.34863271199 3512.88782084123 3427.50612031721 3343.16673453836 3259.83405191936 3177.4735894952 3096.05193942085 3015.5367181852 2935.89651837023 2857.10086279818 2779.12016091979 2701.92566730665 2625.48944211983 2549.78431343512;4598.50163279235 4494.40823886693 4391.78924195184 4290.59438407447 4190.77517898491 4092.28482510566 3995.07812326983 3899.11139893372 3804.34242857308 3710.73036999313 3618.23569630166 3526.82013331263 3436.44660016381 3347.079152947 3258.68293116342 3171.22410682959 3084.66983607064 2998.98821304921 2914.1482260877 2830.11971585147;5054.00279004754 4939.59850244808 4826.81465715762 4715.59601793749 4605.88929576838 4497.64305317735 4390.80761382767 4285.3349770262 4181.17873682896 4078.2940054479 3976.63734068395 3876.16667713006 3776.84126090677 3678.62158770879 3581.46934395661 3485.34735086099 ...(+2764 chars)]  tireParamSet=vdynPassCar.mat  PRESMAX=1000000  PRESMIN=10000  FZMAX=28000  FZMIN=100  VXLOW=1  KPUMAX=1.5  KPUMIN=-1.5  ALPMAX=1.5  ALPMIN=-1.5  CAMMAX=0.17453  CAMMIN=-0.17453  LONGVL=16.7  FxRelFreqLwrLim=200*pi  FyRelFreqLwrLim=200*pi  MyRelFreqLwrLim=100*pi  omegao=vdb_v0/(0.97*0.5132)  br=1e-3  UNLOADED_RADIUS=0.5132  NOMPRES=793000  FNOMIN=3166.8363806  WIDTH=0.295  RIM_RADIUS=0.28575  MASS=54.96  IYY=10.664  GRAVITY=-9.81  zo=0  zdoto=0  BREFF=8.25094594147963  DREFF=0.260468730454265  FREFF=0.0735298544471851  Q_RE0=1.00866439868088  Q_V1=0.000760413786224011  Q_V2=0.0463384792019201  Q_FZ1=0  Q_FZ2=15.6870832810226  Q_FZ3=0  Q_FCX=0.138643970247602  Q_FCY=0.10843499565426  Q_FCY2=-0.465763352339538  PFZ1=0.69958166705601  VERTICAL_STIFFNESS=207885.061134007  VERTICAL_DAMPING=500  BOTTOM_OFFST=.01  BOTTOM_STIFF=2e6  LONGITUDINAL_STIFFNESS=388714.175879854  LATERAL_STIFFNESS=157087.404633332  PCFX1=0.18539229191199  PCFX2=0  PCFX3=0  PCFY1=0.163183345037677  PCFY2=0  PCFY3=0.249094918231954  Q_RA1=0.675942571700787  Q_RA2=0.73800463546164  Q_RB1=1.04487486456705  Q_RB2=-1.191763806629  PCX1=1.58523057950359  PDX1=1.0239116238178  PDX2=-0.0842405110022724  PDX3=0  PEX1=0.110312777158455  PEX2=0.313468516038146  PEX3=0  PEX4=0.0016060905760045  PKX1=21.3872544684023  PKX2=14.0006541873175  PKX3=-0.405326109653452  PHX1=0.000212599305364818  PHX2=0.00115950515263055  PVX1=1.59236164471432e-05  PVX2=0.000104321112127671  PPX1=-0.349461321276586  PPX2=0.387840040616429  PPX3=-0.0969947336569324  PPX4=0.0632271859795801  RBX1=12.7633329850276  RBX2=9.5787123658471  RBX3=0  RCX1=1.02796280922059  REX1=-0.45202516851367  REX2=-0.47304886171176  RHX1=0.000233272373115809  QSX1=-0.00788307788961443  QSX2=0.954629515459396  QSX3=0.0155855777667025  QSX4=0.125904607142414  QSX5=1.01110069703963  QSX6=20.1938577118433  QSX7=0.310818120717083  QSX8=-0.0430823751139655  QSX9=0.636494404888216  QSX10=0.142438060591663  QSX11=0.346766530036373  QSX12=0  QSX13=0  QSX14=0  PPMX1=0  PCY1=1.3  PDY1=1  PDY2=0  PDY3=0  PEY1=-1  PEY2=0  PEY3=0  PEY4=0  PEY5=0  PKY1=-25.2618040168  PKY2=1  PKY3=0  PKY4=2  PKY5=0  PKY6=0  PKY7=0  PHY1=0  PHY2=0  PVY1=0  PVY2=0  PVY3=0  PVY4=0  PPY1=0  PPY2=0  PPY3=0  PPY4=0  PPY5=0  RBY1=0  RBY2=0  RBY3=0  RBY4=0  RCY1=1  REY1=0  REY2=0  RHY1=0  RHY2=0  RVY1=0  RVY2=0  RVY3=0  RVY4=0  RVY5=0  RVY6=0  QSY1=0  QSY2=0  QSY3=0  QSY4=0  QSY5=0  QSY6=0  QSY7=0  QSY8=0  QBZ1=11.666656027484  QBZ2=-1.30355438574485  QBZ3=0  QBZ4=0.177918305399071  QBZ5=-0.162481135068033  QBZ6=0  QBZ9=30.1445534682089  QBZ10=0  QCZ1=1.29026978207574  QDZ1=0.0886972644991399  QDZ2=-0.0058634820161856  QDZ3=0.3805597481383  QDZ4=0  QDZ6=0.00160914918118959  QDZ7=-0.00211036330862154  QDZ8=-0.13921904912557  QDZ9=0.00816585550028243  QDZ10=0  QDZ11=0  QEZ1=-2.19802254534746  QEZ2=1.01850535789165  QEZ3=0  QEZ4=0.278379679112054  QEZ5=-0.548414722765386  QHZ1=0.00148361198869669  QHZ2=0.00202017567585904  QHZ3=0.240316641332066  QHZ4=-0.210114035738085  PPZ1=-0.443927982388615  PPZ2=0  SSZ1=0.00914999585397887  SSZ2=0.0389830656052735  SSZ3=0  SSZ4=0  PDXP1=0.396718274678791  PDXP2=0  PDXP3=0  PKYP1=1.00587060633573  PDYP1=0.40483048923438  PDYP2=0  PDYP3=0  PDYP4=0  PHYP1=0.992731942067188  PHYP2=0.150352945499914  PHYP3=0  PHYP4=-3.98988682633674  PECP1=0.502379254513503  PECP2=0  QDTP1=10.0178654287947  QCRP1=0.200627747200702  QCRP2=0.0995735881599772  QBRP1=0.0997107127960717  QDRP1=1.01432910167423  QDRP2=0  aMode=2
  TrCalc : MATLAB Function  TreatAsAtomicUnit=on
  c1_AxlTrq : Constant  Value=0
  c1_BrkPrs : Constant  Value=0
  c1_Camber : Constant  Value=0
  c1_Fext : Constant  Value=4548.7286194
  c1_Gnd : Constant  Value=0
  c1_Prs : Constant  Value=220000
  c1_YawRate : Constant  Value=0
  c2_AxlTrq : Constant  Value=0
  c2_BrkPrs : Constant  Value=0
  c2_Camber : Constant  Value=0
  c2_Fext : Constant  Value=3166.8363806
  c2_Gnd : Constant  Value=0
  c2_Prs : Constant  Value=220000
  c2_YawRate : Constant  Value=0
  in_a : Constant  Value=l_f
  in_b : Constant  Value=l_r
  in_n : Constant  Value=n_st
  mu_vec1 : Gain  Gain=[0;0;1;0;zeros(23,1)]  Multiplication=Matrix(K*u)
  mu_vec2 : Gain  Gain=[0;0;1;0;zeros(23,1)]  Multiplication=Matrix(K*u)
  sf_base1 : Constant  Value=[1;1;0;0;ones(23,1)]
  sf_base2 : Constant  Value=[1;1;0;0;ones(23,1)]
  sf_sum1 : Sum
  sf_sum2 : Sum
  trc1 : Constant  Value=e_p0
  trc2 : Constant  Value=t_0
  trc3 : Constant  Value=C_alpha_f
  trc4 : Constant  Value=F_zf
  trc5 : Constant  Value=n_st
  F_yf : Outport
  F_yr : Outport  Port=2
  T_r : Outport  Port=3
  wires:
  Tire_rear/8 -> Term_t2_8/1
  Tire_rear/7 -> Term_t2_7/1
  Tire_rear/6 -> Term_t2_6/1
  Tire_rear/5 -> Term_t2_5/1
  Tire_rear/3 -> Term_t2_3/1
  Tire_rear/2 -> Term_t2_2/1
  Tire_rear/1 -> Term_t2_1/1
  Tire_front/8 -> Term_t1_8/1
  Tire_front/7 -> Term_t1_7/1
  Tire_front/6 -> Term_t1_6/1
  Tire_front/5 -> Term_t1_5/1
  Tire_front/3 -> Term_t1_3/1
  Tire_front/2 -> Term_t1_2/1
  Tire_front/1 -> Term_t1_1/1
  TrCalc/1(Tr) -> T_r/1
  TireInputs/5(alF) -> TrCalc/1(alF)
  trc5/1 -> TrCalc/8(n)
  trc4/1 -> TrCalc/7(Fzf)
  trc3/1 -> TrCalc/6(Ca)
  trc2/1 -> TrCalc/5(t0)
  trc1/1 -> TrCalc/4(ep0)
  Gain_F2/1 -> F_yr/1
  Tire_rear/4 -> Gain_F2/1
  Gain_F1/1 -> TrCalc/2(Fyf), F_yf/1
  Tire_front/4 -> Gain_F1/1
  TireInputs/4(VyR) -> Tire_rear/4
  TireInputs/3(VxR) -> Tire_rear/3
  TireInputs/2(VyF) -> Tire_front/4
  TireInputs/1(VxF) -> Tire_front/3
  sf_sum2/1 -> Tire_rear/10
  mu_vec2/1 -> sf_sum2/2
  sf_base2/1 -> sf_sum2/1
  c2_Fext/1 -> Tire_rear/9
  c2_Gnd/1 -> Tire_rear/8
  c2_Prs/1 -> Tire_rear/7
  c2_YawRate/1 -> Tire_rear/6
  c2_Camber/1 -> Tire_rear/5
  c2_AxlTrq/1 -> Tire_rear/2
  c2_BrkPrs/1 -> Tire_rear/1
  sf_sum1/1 -> Tire_front/10
  mu_vec1/1 -> sf_sum1/2
  sf_base1/1 -> sf_sum1/1
  mu/1 -> TrCalc/3(mu), mu_vec2/1, mu_vec1/1
  c1_Fext/1 -> Tire_front/9
  c1_Gnd/1 -> Tire_front/8
  c1_Prs/1 -> Tire_front/7
  c1_YawRate/1 -> Tire_front/6
  c1_Camber/1 -> Tire_front/5
  c1_AxlTrq/1 -> Tire_front/2
  c1_BrkPrs/1 -> Tire_front/1
  in_n/1 -> TireInputs/7(n)
  in_b/1 -> TireInputs/6(b)
  in_a/1 -> TireInputs/5(a)
  v/1 -> TireInputs/4(v)
  gamma/1 -> TireInputs/3(gamma)
  beta/1 -> TireInputs/2(beta)
  theta2/1 -> TireInputs/1(theta2)

== system Model_MapPID_VDBTire/Model_MapPID/Reference_true/Cal T_d_ref ==
  v : Inport
  a_y : Inport  Port=2
  Abs_ay : Abs  SaturateOnIntegerOverflow=off
  LUT_Tdref : Lookup_n-D  BreakpointsForDimension1=Tdref_v_bp_ms  BreakpointsForDimension2=Tdref_ay_bp_ms2  Table=Tdref_table  ExtrapMethod=Clip  InternalRulePriority=Speed  RndMeth=Simplest
      settings: InputPortMap=u0,u1
  Prod_Tdref : Product  Inputs=**
  Sign_ay : Signum
  T_d_ref : Outport
  wires:
  Prod_Tdref/1 -> T_d_ref/1
  Sign_ay/1 -> Prod_Tdref/2
  LUT_Tdref/1 -> Prod_Tdref/1
  [a_y] -> Sign_ay/1
  Abs_ay/1 -> LUT_Tdref/2
  [a_y] -> Abs_ay/1
  v/1 -> LUT_Tdref/1
  a_y/1 -> [a_y]

== system Model_MapPID_VDBTire/Model_MapPID/MapPID/Reference/Cal T_d_ref ==
  v : Inport
  a_y : Inport  Port=2
  Abs_ay : Abs  SaturateOnIntegerOverflow=off
  LUT_Tdref : Lookup_n-D  BreakpointsForDimension1=Tdref_v_bp_ms  BreakpointsForDimension2=Tdref_ay_bp_ms2  Table=Tdref_table  ExtrapMethod=Clip  InternalRulePriority=Speed  RndMeth=Simplest
      settings: InputPortMap=u0,u1
  Prod_Tdref : Product  Inputs=**
  Sign_ay : Signum
  T_d_ref : Outport
  wires:
  a_y/1 -> [a_y]
  v/1 -> LUT_Tdref/1
  [a_y] -> Abs_ay/1
  Abs_ay/1 -> LUT_Tdref/2
  [a_y] -> Sign_ay/1
  LUT_Tdref/1 -> Prod_Tdref/1
  Sign_ay/1 -> Prod_Tdref/2
  Prod_Tdref/1 -> T_d_ref/1

== system Model_MapPID_VDBTire/Model_MapPID/Plant/Bike2DOF/Beta ==
  F_sum : Inport
  v : Inport  Port=2
  gamma : Inport  Port=3
  Constant : Constant  Value=m
  Div_Fsum_mv : Product  Inputs=*/
  Int_beta : Integrator
  Prod_mv : Product  Inputs=**
  Sum_betadot : Sum  Inputs=+-
  beta : Outport
  wires:
  Int_beta/1 -> beta/1
  Sum_betadot/1 -> Int_beta/1
  gamma/1 -> Sum_betadot/2
  Div_Fsum_mv/1 -> Sum_betadot/1
  Prod_mv/1 -> Div_Fsum_mv/2
  F_sum/1 -> Div_Fsum_mv/1
  v/1 -> Prod_mv/2
  Constant/1 -> Prod_mv/1

== system Model_MapPID_VDBTire/Model_MapPID/Plant/Bike2DOF/Cal Fsum ==
  F_yf : Inport
  F_yr : Inport  Port=2
  Sum_Fsum : Sum
  F_sum : Outport
  wires:
  Sum_Fsum/1 -> F_sum/1
  F_yr/1 -> Sum_Fsum/2
  F_yf/1 -> Sum_Fsum/1

== system Model_MapPID_VDBTire/Model_MapPID/Plant/Bike2DOF/Cal a_y ==
  F_sum : Inport
  Constant : Constant  Value=m
  Div_ay : Product  Inputs=*/
  a_y : Outport
  wires:
  Div_ay/1 -> a_y/1
  Constant/1 -> Div_ay/2
  F_sum/1 -> Div_ay/1

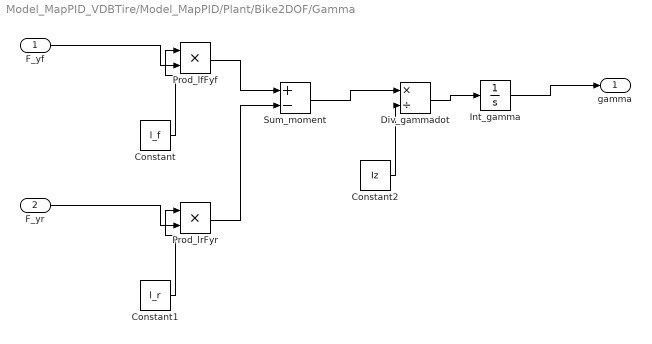
== system Model_MapPID_VDBTire/Model_MapPID/Plant/Bike2DOF/Gamma ==
  F_yf : Inport
  F_yr : Inport  Port=2
  Constant : Constant  Value=l_f
  Constant1 : Constant  Value=l_r
  Constant2 : Constant  Value=Iz
  Div_gammadot : Product  Inputs=*/
  Int_gamma : Integrator
  Prod_lfFyf : Product  Inputs=**
  Prod_lrFyr : Product  Inputs=**
  Sum_moment : Sum  Inputs=+-
  gamma : Outport
  wires:
  Int_gamma/1 -> gamma/1
  Div_gammadot/1 -> Int_gamma/1
  Constant2/1 -> Div_gammadot/2
  Sum_moment/1 -> Div_gammadot/1
  Prod_lrFyr/1 -> Sum_moment/2
  Prod_lfFyf/1 -> Sum_moment/1
  F_yr/1 -> Prod_lrFyr/2
  Constant1/1 -> Prod_lrFyr/1
  F_yf/1 -> Prod_lfFyf/2
  Constant/1 -> Prod_lfFyf/1

== system Model_MapPID_VDBTire/Model_MapPID/Plant/SteeringColumn/Cal T_s ==
  theta1 : Inport
  theta2 : Inport  Port=2
  Constant : Constant  Value=K
  Prod_Ts : Product  Inputs=**
  Sum_dTheta : Sum  Inputs=+-
  T_s : Outport
  wires:
  Prod_Ts/1 -> T_s/1
  Constant/1 -> Prod_Ts/2
  Sum_dTheta/1 -> Prod_Ts/1
  theta2/1 -> Sum_dTheta/2
  theta1/1 -> Sum_dTheta/1

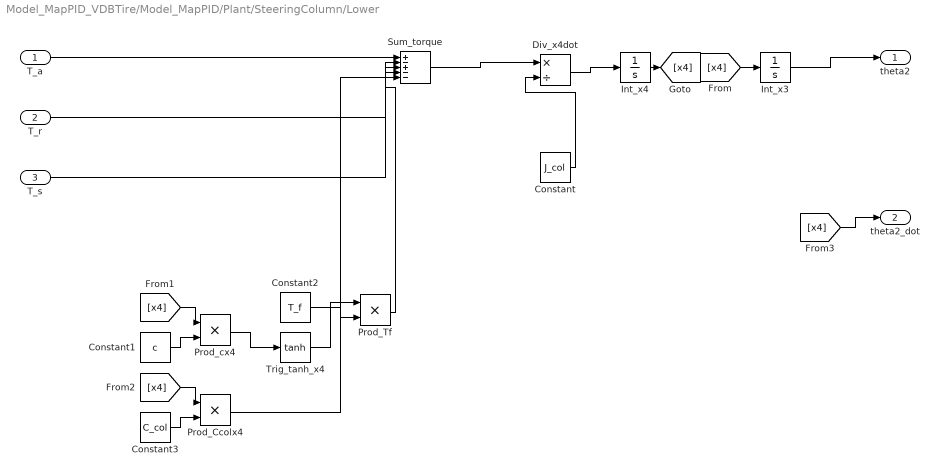
== system Model_MapPID_VDBTire/Model_MapPID/Plant/SteeringColumn/Lower ==
  T_a : Inport
  T_r : Inport  Port=2
  T_s : Inport  Port=3
  Constant : Constant  Value=J_col
  Constant1 : Constant  Value=c
  Constant2 : Constant  Value=T_f
  Constant3 : Constant  Value=C_col
  Div_x4dot : Product  Inputs=*/
  Int_x3 : Integrator
  Int_x4 : Integrator
  Prod_Ccolx4 : Product  Inputs=**
  Prod_Tf : Product  Inputs=**
  Prod_cx4 : Product  Inputs=**
  Sum_torque : Sum  Inputs=+-+--
  Trig_tanh_x4 : Trigonometry  Operator=tanh
  theta2 : Outport
  theta2_dot : Outport  Port=2
  wires:
  [x4] -> theta2_dot/1
  Int_x3/1 -> theta2/1
  [x4] -> Int_x3/1
  Div_x4dot/1 -> Int_x4/1
  Constant/1 -> Div_x4dot/2
  Sum_torque/1 -> Div_x4dot/1
  Prod_Ccolx4/1 -> Sum_torque/5
  Prod_Tf/1 -> Sum_torque/4
  T_s/1 -> Sum_torque/3
  T_r/1 -> Sum_torque/2
  T_a/1 -> Sum_torque/1
  Constant3/1 -> Prod_Ccolx4/2
  [x4] -> Prod_Ccolx4/1
  Constant2/1 -> Prod_Tf/2
  Trig_tanh_x4/1 -> Prod_Tf/1
  Prod_cx4/1 -> Trig_tanh_x4/1
  Constant1/1 -> Prod_cx4/2
  [x4] -> Prod_cx4/1
  Int_x4/1 -> [x4]

== matlab function Model_MapPID_VDBTire/Model_MapPID/Plant/Tires/TrCalc ==
  data: alF input; Tr output; Fyf input; mu input; ep0 input; t0 input; Ca input; Fzf input; n input
function Tr = f(alF, Fyf, mu, ep0, t0, Ca, Fzf, n)
ec = ep0 - t0;
ep = ec + max(0, t0 - sign(alF)*t0*Ca*tan(alF)/(3*mu*Fzf));   % pneumatic trail
Tr = ep/n*Fyf;

== matlab function Model_MapPID_VDBTire/Model_MapPID/Plant/Tires/TireInputs ==
  data: theta2 input; VxF output; beta input; gamma input; v input; a input; b input; n input; VyF output; VxR output; VyR output; alF output
function [VxF, VyF, VxR, VyR, alF] = f(theta2, beta, gamma, v, a, b, n)
alF = theta2/n - beta - a*gamma/v;     % Plant (10), delta_f = theta2/n_st
alR = -beta + b*gamma/v;               % Plant (11)
VxF = v; VyF = -v*tan(alF);            % VDB alpha = atan(Vy/Vx) = -alpha_f
VxR = v; VyR = -v*tan(alR);
